simulink model "LinearRLStability"  (R2025a)
settings: Solver=ode15s  StartTime=0.0  StopTime=0.1  RelTol=1e-3
settings Model: Creator=matthiasmees  LastModifiedBy=matthiasmees
settings DataIOCC: ReturnWorkspaceOutputs=off

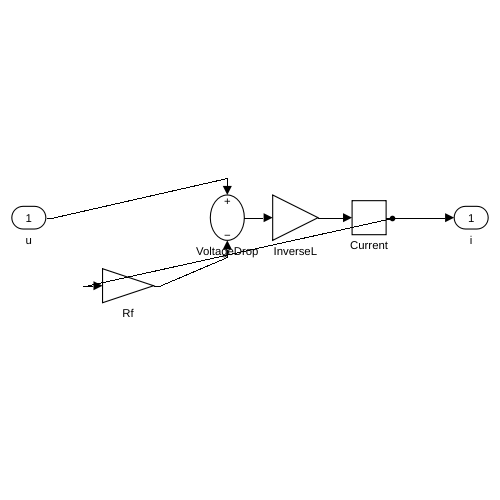
[thumbnail: Simulink's stored preview of the top-level diagram]
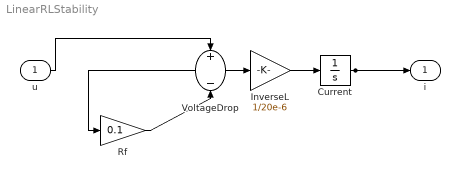
== system LinearRLStability ==
  u : Inport
  Current : Integrator
  InverseL : Gain  Gain=1/20e-6
  Rf : Gain  Gain=0.1
  VoltageDrop : Sum  Inputs=+-
  i : Outport
  wires:
  u/1 -> VoltageDrop/1
  Current/1 -> Rf/1, i/1
  Rf/1 -> VoltageDrop/2
  VoltageDrop/1 -> InverseL/1
  InverseL/1 -> Current/1
